simulink model "boost_simscape_R2021b"  (R2021b)
settings: Solver=FixedStepDiscrete  StartTime=0  StopTime=(N-1)*Ts  FixedStep=h  RelTol=1e-3
model workspace (MAT data in the model file):
  CP = [2 0.03 20 0 0 1 0 0 0.15 12 12 48 0.5 0.05 0.9 0.0005 5e-05 0 60 0 18 0 15 0 60 24 0 0 0 0 0 0]
  Cp = 0.00047
  D0 = 0.5
  Gdp = 1e-08
  LP = [1 0.05 20 10 0 0 0]
  Lp = 0.0005
  N = 2000
  OL = 0
  Rdp = 0.0001
  Roff_sw = 1000000
  Ron_sw = 0.001
  Ts = 5e-05
  VP = [0 24 0 0 0 0 0]
  Vfp = 1e-06
  X0 = [0; 0; 0; 0; 0; 0.5; 0.5; 0.5]
  cpk = 0.999999999
  d_ol = 0
  fine_dec = 1
  h = 1e-07
  iL0p = 0
  rCp = 1e-06
  rLp = 0
  vC0p = 24
libraries: nesl_utility x7, simulink x1
settings Model: Creator=runner  LastModifiedBy=runner
settings DebuggingCC: AlgebraicLoopMsg=error  UnconnectedInputMsg=none  UnconnectedOutputMsg=none  UnconnectedLineMsg=none
settings ModelReferenceCC: EnableRefExpFcnMdlSchedulingChecks=off
settings RTWCC: DLArmComputeVersion=20.02.1

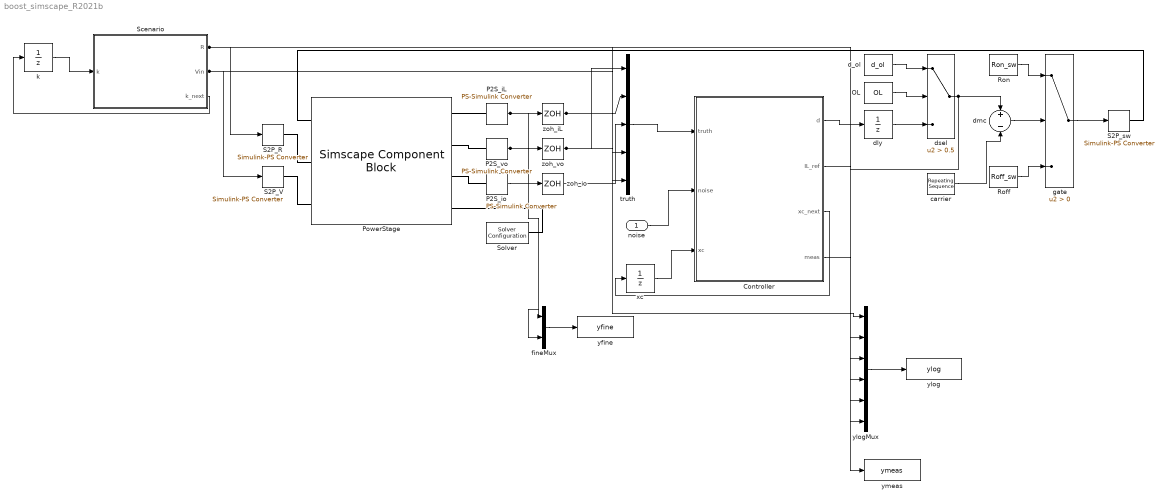
== system boost_simscape_R2021b ==
  noise : Inport  PortDimensions=4  SampleTime=Ts
  Controller : MATLAB Function  TreatAsAtomicUnit=on
  OL : Constant  Value=OL
  P2S_iL : nesl_utility/PS-Simulink Converter  PhysicalDomain=network_engine_domain  SubClassName=ps_output  LeftPortType=input  RightPortType=output  PseudoPeriodic=off  Frequencies=[]  VectorFormat=inherit  Unit=A  AffineConversion=off
  P2S_io : nesl_utility/PS-Simulink Converter  PhysicalDomain=network_engine_domain  SubClassName=ps_output  LeftPortType=input  RightPortType=output  PseudoPeriodic=off  Frequencies=[]  VectorFormat=inherit  Unit=A  AffineConversion=off
  P2S_vo : nesl_utility/PS-Simulink Converter  PhysicalDomain=network_engine_domain  SubClassName=ps_output  LeftPortType=input  RightPortType=output  PseudoPeriodic=off  Frequencies=[]  VectorFormat=inherit  Unit=V  AffineConversion=off
  PowerStage : SimscapeComponentBlock  SourceFile=boost_stage  ComponentPath=boost_stage  ComponentVariants="[\"boost_stage\"]"  ComponentVariantNames="[\"boost_stage\"]"  ClassName=boost_stage  SchemaVersion=1  L=Lp H  rL=rLp Ohm  C=Cp F  rC=rCp Ohm  Vf=Vfp V  Rd=Rdp Ohm  Gd=Gdp 1/Ohm  iL0=iL0p A  vC0=vC0p V
      settings: CopyFcn=simscape.engine.sli.internal.componentblockcallback(gcbh,'COPY')  PreCopyFcn=simscape.engine.sli.internal.componentblockcallback(gcbh,'PRECOPY')  PreDeleteFcn=simscape.engine.sli.internal.componentblockcallback(gcbh,'PREDELETE')  InternalSimscapePortConfiguration="{\"Bottom\":[],\"Left\":[{\"id\":\"Rsw\",\"label\":\"Rsw\",\"type\":\"input\"},{\"id\":\"Rload\",\"label\":\"Rload\",\"type\":\"input\"},{\"id\":\"Vin\",\"label\":\"Vin\",\"type\":\"input\"}],\"Right\":[{\"id\":\"iL\",\"label\":\"iL\",\"type\":\"output\"},{\"id\":\"vo\",\"label\":\"vo\",\"type\":\"output\"},{\"id\":\"io\",\"label\":\"io\",\"type\":\"output\"},{\"id\":\"g\",\"label\":\"G\",\"type\":\"foundation.electrical.electrical\"}],\"Top\":[]}"
      mask Type: Boost power stage (Simscape Foundation blocks)
  Roff : Constant  Value=Roff_sw
  Ron : Constant  Value=Ron_sw
  S2P_R : nesl_utility/Simulink-PS Converter  PhysicalDomain=network_engine_domain  SubClassName=ps_input  LeftPortType=input  RightPortType=output  PseudoPeriodic=off  Frequencies=[]  NoiseDistribution=none  NoiseParameters=[]  Unit=Ohm  AffineConversion=off  FilteringAndDerivatives=provide  SimscapeFilterOrder=1  InputFilterTimeConstant=0.001  UdotUserProvided=0
  S2P_V : nesl_utility/Simulink-PS Converter  PhysicalDomain=network_engine_domain  SubClassName=ps_input  LeftPortType=input  RightPortType=output  PseudoPeriodic=off  Frequencies=[]  NoiseDistribution=none  NoiseParameters=[]  Unit=V  AffineConversion=off  FilteringAndDerivatives=provide  SimscapeFilterOrder=1  InputFilterTimeConstant=0.001  UdotUserProvided=0
  S2P_sw : nesl_utility/Simulink-PS Converter  PhysicalDomain=network_engine_domain  SubClassName=ps_input  LeftPortType=input  RightPortType=output  PseudoPeriodic=off  Frequencies=[]  NoiseDistribution=none  NoiseParameters=[]  Unit=Ohm  AffineConversion=off  FilteringAndDerivatives=provide  SimscapeFilterOrder=1  InputFilterTimeConstant=0.001  UdotUserProvided=0
  Scenario : MATLAB Function  TreatAsAtomicUnit=on
  Solver : nesl_utility/Solver Configuration  PhysicalDomain=network_engine_domain  SubClassName=solver  LeftPortType=input  RightPortType=generic  Tones=[]  Harmonics=[]  SimulateNoise=off  Profile=off  UseLocalSampling=off  EnableSwitchedLinearOptims=on  FrequencyDomain=off  UseCCode=off  RelTol=0.001  AbsTol=0.001  MinStep=1e-09  ToWorkspace=off  RevertToSquareIcSolve=off  NumHomotopyIterations=100  PhasorMode=off  PhasorModeNumHarmonics=1  ConsistencySolver=NEWTON_XTOL_AFTER_FTOL  IndexReductionMethod=DerivativeReplacement  DoDC=off  ResidualTolerance=1e-09  ConsistencyTolSource=GLOBAL  ConsistencyAbsTol=0.001  ConsistencyRelTol=0.001  ConsistencyTolFactor=0.001  UseLocalSolver=on  LocalSolverChoice=NE_BACKWARD_EULER_ADVANCER  ResolveIndetEquations=on  FunctionEvalNumThread=1  LocalSolverSampleTime=h  DoFixedCost=off  MaxNonlinIter=20  MaxModeIter=20  ComputeImpulses=off  ImpulseIterations=2  LinearAlgebra=auto  LinearAlgebraNumThread=0  EquationFormulation=NE_TIME_EF  DelaysMemoryBudget=1024  AutomaticFiltering=on  FilteringTimeConstant=0.001  PartitionStorageMethod=AS_NEEDED  PartitionMemoryBudget=1024  PartitionMethod=ROBUST  MultibodyUseLocalSolver=off  MultibodyLocalSolverChoice=ODE1  MultibodyLocalSolverSampleTime=0.001
  carrier : simulink/Sources/Repeating Sequence  rep_seq_t=[0 h/2 Ts/2+h/2 Ts]  rep_seq_y=[cpk*h/Ts 0 cpk cpk*h/Ts]
  d_ol : Constant  Value=d_ol
  dly : UnitDelay  InitialCondition=D0  SampleTime=Ts  HasFrameUpgradeWarning=on
  dmc : Sum  Inputs=+-
  dsel : Switch  Criteria=u2 > Threshold  Threshold=0.5
  fineMux : Mux  Inputs=2
  gate : Switch  Criteria=u2 > Threshold
  k : UnitDelay  SampleTime=Ts  HasFrameUpgradeWarning=on
  truth : Mux  Inputs=5
  xc : UnitDelay  InitialCondition=X0  SampleTime=Ts  HasFrameUpgradeWarning=on
  yfine : ToWorkspace  VariableName=yfine  SampleTime=-1
      settings: Decimation=fine_dec
  ylog : ToWorkspace  VariableName=ylog  SampleTime=Ts
  ylogMux : Mux  Inputs=6
  ymeas : ToWorkspace  VariableName=ymeas  SampleTime=Ts
  zoh_iL : ZeroOrderHold  SampleTime=Ts
  zoh_io : ZeroOrderHold  SampleTime=Ts
  zoh_vo : ZeroOrderHold  SampleTime=Ts
  wires:
  k/1 -> Scenario/1(k)
  Scenario/3(k_next) -> k/1
  Scenario/1(R) -> S2P_R/1, truth/5, ylogMux/5
  Scenario/2(Vin) -> S2P_V/1, truth/4, ylogMux/6
  P2S_iL/1 -> zoh_iL/1, fineMux/1
  P2S_vo/1 -> zoh_vo/1, fineMux/2
  P2S_io/1 -> zoh_io/1
  zoh_vo/1 -> truth/1, ylogMux/1
  zoh_iL/1 -> truth/2, ylogMux/2
  zoh_io/1 -> truth/3
  truth/1 -> Controller/1(truth)
  noise/1 -> Controller/2(noise)
  xc/1 -> Controller/3(xc)
  Controller/3(xc_next) -> xc/1
  Controller/1(d) -> dly/1
  d_ol/1 -> dsel/1
  OL/1 -> dsel/2
  dly/1 -> dsel/3
  dsel/1 -> dmc/1, ylogMux/3
  carrier/1 -> dmc/2
  Ron/1 -> gate/1
  dmc/1 -> gate/2
  Roff/1 -> gate/3
  gate/1 -> S2P_sw/1
  Controller/2(IL_ref) -> ylogMux/4
  ylogMux/1 -> ylog/1
  Controller/4(meas) -> ymeas/1
  fineMux/1 -> yfine/1
  connections:
  S2P_sw/RConn1 -- PowerStage/LConn1
  S2P_R/RConn1 -- PowerStage/LConn2
  S2P_V/RConn1 -- PowerStage/LConn3
  PowerStage/RConn1 -- P2S_iL/LConn1
  PowerStage/RConn2 -- P2S_vo/LConn1
  PowerStage/RConn3 -- P2S_io/LConn1
  PowerStage/RConn4 -- Solver/RConn1

== matlab function boost_simscape_R2021b/Controller ==
  settings: updateMethod=DISCRETE  sampleTime=Ts
  data: truth input; d output; noise input; xc input double size=[8 1]; IL_ref output; xc_next output; meas output; CP parameter
function [d, IL_ref, xc_next, meas] = ctrl(truth, noise, xc, CP)
[d, IL_ref, xc_next, meas] = blk_controller(truth, noise, xc, CP);
end

== matlab function boost_simscape_R2021b/Scenario ==
  settings: updateMethod=DISCRETE  sampleTime=Ts
  data: k input double size=1; R output; Vin output; k_next output; LP parameter; VP parameter; Ts parameter
function [R, Vin, k_next] = scen(k, LP, VP, Ts)
[R, Vin, k_next] = blk_scenario(k, LP, VP, Ts);
end
